simulink model "InvertedPendulum_LQR_Controller"  (R2023a)
settings: Solver=ode4  StartTime=0.0  StopTime=5  FixedStep=0.001  RelTol=1e-3
settings Model: Creator=Fasih  LastModifiedBy=Fasih

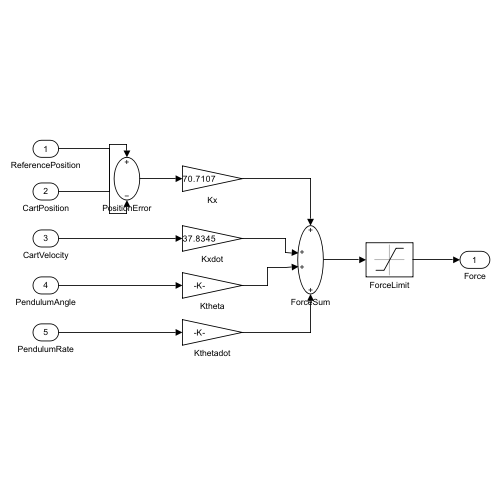
[thumbnail: Simulink's stored preview of the top-level diagram]
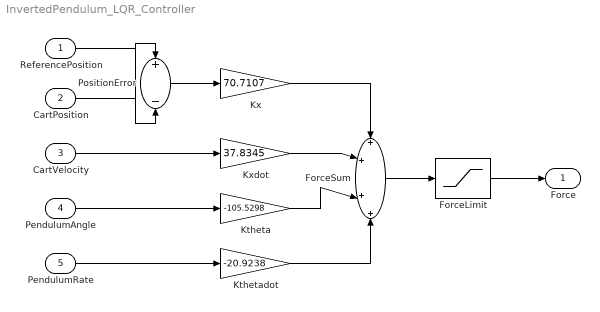
== system InvertedPendulum_LQR_Controller ==
  ReferencePosition : Inport
  CartPosition : Inport  Port=2
  CartVelocity : Inport  Port=3
  PendulumAngle : Inport  Port=4
  PendulumRate : Inport  Port=5
  ForceLimit : Saturate  UpperLimit=10  LowerLimit=-10
  ForceSum : Sum  Inputs=++++
  Ktheta : Gain  Gain=-105.5298
  Kthetadot : Gain  Gain=-20.9238
  Kx : Gain  Gain=70.7107
  Kxdot : Gain  Gain=37.8345
  PositionError : Sum  Inputs=+-
  Force : Outport
  wires:
  CartPosition/1 -> PositionError/1
  ReferencePosition/1 -> PositionError/2
  PositionError/1 -> Kx/1
  CartVelocity/1 -> Kxdot/1
  PendulumAngle/1 -> Ktheta/1
  PendulumRate/1 -> Kthetadot/1
  Kx/1 -> ForceSum/1
  Kxdot/1 -> ForceSum/2
  Ktheta/1 -> ForceSum/3
  Kthetadot/1 -> ForceSum/4
  ForceSum/1 -> ForceLimit/1
  ForceLimit/1 -> Force/1
